simulink subsystem "Othonormalise"  (R2024b)
settings: Solver=VariableStepAuto  StartTime=0.0  StopTime=10.0  RelTol=1e-3
settings Model: Creator=marco  LastModifiedBy=ferru

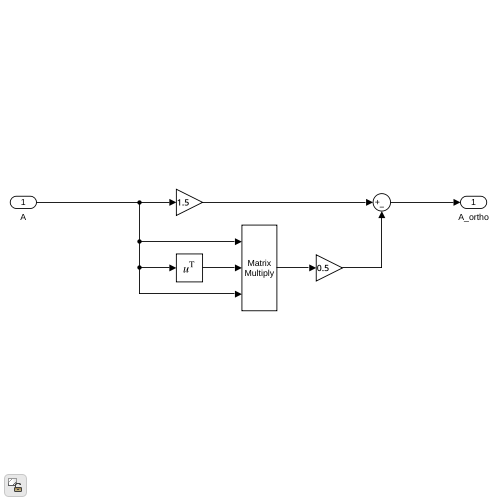
[thumbnail: Simulink's stored preview of the top-level diagram]
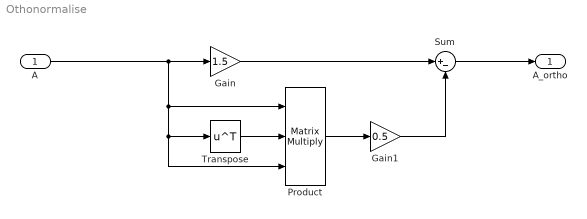
== system Othonormalise ==
  A : Inport
  Gain : Gain  Gain=1.5
  Gain1 : Gain  Gain=0.5
  Product : Product  Inputs=3  Multiplication=Matrix(*)
  Sum : Sum  Inputs=|+-
  Transpose : Math  Operator=transpose
  A_ortho : Outport
  wires:
  Sum/1 -> A_ortho/1
  Gain/1 -> Sum/1
  Transpose/1 -> Product/2
  Product/1 -> Gain1/1
  Gain1/1 -> Sum/2
  A/1 -> Gain/1, Product/3, Transpose/1, Product/1
